simulink model "single_motor_fix"  (R2025b)
settings: Solver=VariableStepAuto  StartTime=0.0  StopTime=10.0  RelTol=1e-3
values from neighbouring files (symbols this model uses):
  Dm = 1e-3    (= 0.001)    [motor_param.m]
  Jm = 0.1e-3    (= 0.0001)    [motor_param.m]
  Ld = 0.01    [motor_param.m]
  Lq = 0.02    [motor_param.m]
  p = 2    [motor_param.m]
  Phi = 0.1    [motor_param.m]
  Rs = 0.38    [motor_param.m]
libraries: fl_lib x20, nesl_utility x20, ee_lib x6, eeTransforms x4, simulink x2
(part 2 of 2)

== matlab function single_motor_fix/Controller/FOC/VelocityController/MATLAB Function ==
  data: w_ref input; u_cmd output; w_m input; bar_w input; xi input; Jm parameter; Dm parameter; dot_bar_w output; dot_xi output
function [u_cmd, dot_bar_w, dot_xi] = FixedTimeController(w_ref, w_m, bar_w, xi, Jm, Dm)

    lambda1  = 5;   lambda2 = 5;   lambda3 = 6;
    tau      = 0.5; vartheta = 1.5;
    k_w = 6; k1 = 5; k2 = 5;

    k_i = 20;

    kappa0 = 30;     % 线性积分增益（新增，压制小误差）
    kappa1 = 20;     % 固定时间项增益
    kappa2 = 20;
    alpha1 = 0.5;
    alpha2 = 1.5;

    pow_func = @(x, gamma) abs(x)^gamma * sign(x);

    % 公式(117) 滤波器
    e_w = bar_w - w_ref;
    dot_bar_w = (1/tau) * ( -lambda1 * pow_func(e_w, 0.5) ...
                            -lambda2 * pow_func(e_w, vartheta) ...
                            -lambda3 * e_w );

    s   = w_m - bar_w;
    e_v = w_m - w_ref;

    % 混合固定时间积分
    dot_xi = kappa0 * e_v ...
           + kappa1 * pow_func(e_v, alpha1) ...
           + kappa2 * pow_func(e_v, alpha2);

    TL_hat_int = k_i * xi;

    feedback = -k_w * s ...
               - k1 * pow_func(s, 0.5) ...
               - k2 * pow_func(s, vartheta);

    u_cmd = Jm * dot_bar_w + Dm * bar_w - TL_hat_int + feedback;
end
